simulink model "asm_blocks_lib"  (R2026b)
settings: Solver=VariableStepAuto
libraries: nesl_utility x45, asmlib_lib x25, fl_lib x3, ee_lib x3
(part 3 of 3)

== system asm_blocks_lib/Mechanik/Welle elastisch ==
  elastic_shaft : asmlib_lib/mechanics/Elastic shaft  c_W=c_W N*m/rad  d_W=d_W N*m*s/rad  t_specify=off  t_priority=None  t=0 N*m  t_nominal_specify=off  t_nominal_value=1  t_nominal_unit=N*m  w_specify=off  w_priority=None  w=0 rad/s  w_nominal_specify=off  w_nominal_value=1  w_nominal_unit=rad/s  phi_specify=off  phi_priority=High  phi=0 rad  phi_nominal_specify=off  phi_nominal_value=1  phi_nominal_unit=rad
  R : PMIOPort  Side=Left
  C : PMIOPort  Port=2  Side=Right
  connections:
  R/RConn1 -- elastic_shaft/LConn1
  C/RConn1 -- elastic_shaft/RConn1

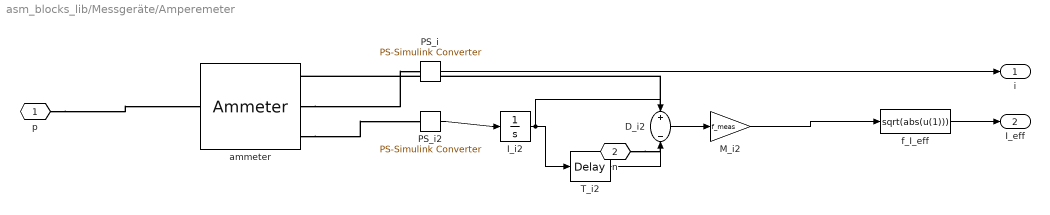
== system asm_blocks_lib/Messgeräte/Amperemeter ==
  D_i2 : Sum  Inputs=+-
  I_i2 : Integrator
  M_i2 : Gain  Gain=f_meas
  PS_i : nesl_utility/PS-Simulink Converter  PhysicalDomain=network_engine_domain  SubClassName=ps_output  LeftPortType=input  RightPortType=output  PseudoPeriodic=off  Frequencies=[]  VectorFormat=inherit  Unit=A  AffineConversion=off
  PS_i2 : nesl_utility/PS-Simulink Converter  PhysicalDomain=network_engine_domain  SubClassName=ps_output  LeftPortType=input  RightPortType=output  PseudoPeriodic=off  Frequencies=[]  VectorFormat=inherit  Unit=A^2  AffineConversion=off
  T_i2 : TransportDelay  DelayTime=1/f_meas  BufferSize=16384
  ammeter : asmlib_lib/sensors/Ammeter  ii_specify=off  ii_priority=None  ii=0 A  ii_nominal_specify=off  ii_nominal_value=1  ii_nominal_unit=A
  f_I_eff : Fcn  Expr=sqrt(abs(u(1)))
  p : PMIOPort  Side=Left
  n : PMIOPort  Port=2  Side=Right
  i : Outport
  I_eff : Outport  Port=2
  wires:
  PS_i/1 -> i/1
  PS_i2/1 -> I_i2/1
  I_i2/1 -> D_i2/1, T_i2/1
  T_i2/1 -> D_i2/2
  D_i2/1 -> M_i2/1
  M_i2/1 -> f_I_eff/1
  f_I_eff/1 -> I_eff/1
  connections:
  p/RConn1 -- ammeter/LConn1
  n/RConn1 -- ammeter/RConn1
  ammeter/RConn2 -- PS_i/LConn1
  ammeter/RConn3 -- PS_i2/LConn1

== system asm_blocks_lib/Messgeräte/Drehmomentmesswelle ==
  PS_M : nesl_utility/PS-Simulink Converter  PhysicalDomain=network_engine_domain  SubClassName=ps_output  LeftPortType=input  RightPortType=output  PseudoPeriodic=off  Frequencies=[]  VectorFormat=inherit  Unit=N*m  AffineConversion=off
  torque_sensor : asmlib_lib/sensors/Torque sensor  t_specify=off  t_priority=None  t=0 N*m  t_nominal_specify=off  t_nominal_value=1  t_nominal_unit=N*m
  R : PMIOPort  Side=Left
  C : PMIOPort  Port=2  Side=Right
  M : Outport
  wires:
  PS_M/1 -> M/1
  connections:
  R/RConn1 -- torque_sensor/LConn1
  C/RConn1 -- torque_sensor/RConn1
  torque_sensor/RConn2 -- PS_M/LConn1

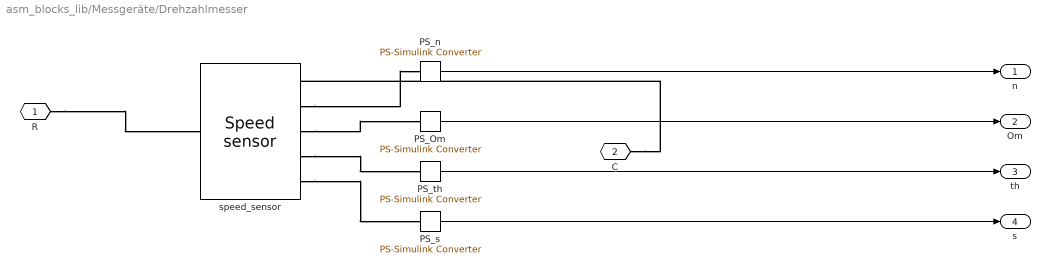
== system asm_blocks_lib/Messgeräte/Drehzahlmesser ==
  PS_Om : nesl_utility/PS-Simulink Converter  PhysicalDomain=network_engine_domain  SubClassName=ps_output  LeftPortType=input  RightPortType=output  PseudoPeriodic=off  Frequencies=[]  VectorFormat=inherit  Unit=rad/s  AffineConversion=off
  PS_n : nesl_utility/PS-Simulink Converter  PhysicalDomain=network_engine_domain  SubClassName=ps_output  LeftPortType=input  RightPortType=output  PseudoPeriodic=off  Frequencies=[]  VectorFormat=inherit  Unit=rpm  AffineConversion=off
  PS_s : nesl_utility/PS-Simulink Converter  PhysicalDomain=network_engine_domain  SubClassName=ps_output  LeftPortType=input  RightPortType=output  PseudoPeriodic=off  Frequencies=[]  VectorFormat=inherit  Unit=1  AffineConversion=off
  PS_th : nesl_utility/PS-Simulink Converter  PhysicalDomain=network_engine_domain  SubClassName=ps_output  LeftPortType=input  RightPortType=output  PseudoPeriodic=off  Frequencies=[]  VectorFormat=inherit  Unit=rad  AffineConversion=off
  speed_sensor : asmlib_lib/sensors/Speed sensor  ns=ns rpm  w_specify=off  w_priority=None  w=0 rad/s  w_nominal_specify=off  w_nominal_value=1  w_nominal_unit=rad/s  ph_specify=off  ph_priority=High  ph=0 rad  ph_nominal_specify=off  ph_nominal_value=1  ph_nominal_unit=rad
  R : PMIOPort  Side=Left
  C : PMIOPort  Port=2  Side=Right
  n : Outport
  Om : Outport  Port=2
  th : Outport  Port=3
  s : Outport  Port=4
  wires:
  PS_n/1 -> n/1
  PS_Om/1 -> Om/1
  PS_th/1 -> th/1
  PS_s/1 -> s/1
  connections:
  R/RConn1 -- speed_sensor/LConn1
  C/RConn1 -- speed_sensor/RConn1
  speed_sensor/RConn2 -- PS_n/LConn1
  speed_sensor/RConn3 -- PS_Om/LConn1
  speed_sensor/RConn4 -- PS_th/LConn1
  speed_sensor/RConn5 -- PS_s/LConn1

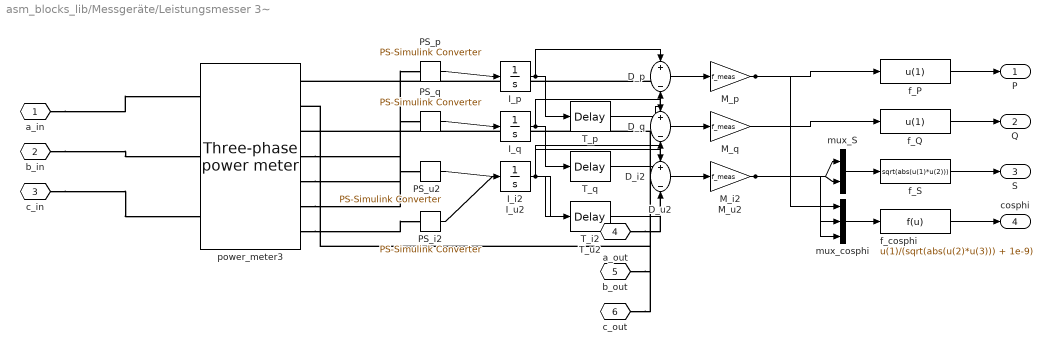
== system asm_blocks_lib/Messgeräte/Leistungsmesser 3~ ==
  D_i2 : Sum  Inputs=+-
  D_p : Sum  Inputs=+-
  D_q : Sum  Inputs=+-
  D_u2 : Sum  Inputs=+-
  I_i2 : Integrator
  I_p : Integrator
  I_q : Integrator
  I_u2 : Integrator
  M_i2 : Gain  Gain=f_meas
  M_p : Gain  Gain=f_meas
  M_q : Gain  Gain=f_meas
  M_u2 : Gain  Gain=f_meas
  PS_i2 : nesl_utility/PS-Simulink Converter  PhysicalDomain=network_engine_domain  SubClassName=ps_output  LeftPortType=input  RightPortType=output  PseudoPeriodic=off  Frequencies=[]  VectorFormat=inherit  Unit=A^2  AffineConversion=off
  PS_p : nesl_utility/PS-Simulink Converter  PhysicalDomain=network_engine_domain  SubClassName=ps_output  LeftPortType=input  RightPortType=output  PseudoPeriodic=off  Frequencies=[]  VectorFormat=inherit  Unit=W  AffineConversion=off
  PS_q : nesl_utility/PS-Simulink Converter  PhysicalDomain=network_engine_domain  SubClassName=ps_output  LeftPortType=input  RightPortType=output  PseudoPeriodic=off  Frequencies=[]  VectorFormat=inherit  Unit=V*A  AffineConversion=off
  PS_u2 : nesl_utility/PS-Simulink Converter  PhysicalDomain=network_engine_domain  SubClassName=ps_output  LeftPortType=input  RightPortType=output  PseudoPeriodic=off  Frequencies=[]  VectorFormat=inherit  Unit=V^2  AffineConversion=off
  T_i2 : TransportDelay  DelayTime=1/f_meas  BufferSize=16384
  T_p : TransportDelay  DelayTime=1/f_meas  BufferSize=16384
  T_q : TransportDelay  DelayTime=1/f_meas  BufferSize=16384
  T_u2 : TransportDelay  DelayTime=1/f_meas  BufferSize=16384
  f_P : Fcn  Expr=u(1)
  f_Q : Fcn  Expr=u(1)
  f_S : Fcn  Expr=sqrt(abs(u(1)*u(2)))
  f_cosphi : Fcn  Expr=u(1)/(sqrt(abs(u(2)*u(3))) + 1e-9)
  mux_S : Mux  Inputs=2
  mux_cosphi : Mux  Inputs=3
  power_meter3 : asmlib_lib/sensors/Three-phase power meter  ia_specify=off  ia_priority=None  ia=0 A  ia_nominal_specify=off  ia_nominal_value=1  ia_nominal_unit=A  ib_specify=off  ib_priority=None  ib=0 A  ib_nominal_specify=off  ib_nominal_value=1  ib_nominal_unit=A  ic_specify=off  ic_priority=None  ic=0 A  ic_nominal_specify=off  ic_nominal_value=1  ic_nominal_unit=A
  a_in : PMIOPort  Side=Left
  b_in : PMIOPort  Port=2  Side=Left
  c_in : PMIOPort  Port=3  Side=Left
  a_out : PMIOPort  Port=4  Side=Right
  b_out : PMIOPort  Port=5  Side=Right
  c_out : PMIOPort  Port=6  Side=Right
  P : Outport
  Q : Outport  Port=2
  S : Outport  Port=3
  cosphi : Outport  Port=4
  wires:
  PS_p/1 -> I_p/1
  I_p/1 -> D_p/1, T_p/1
  T_p/1 -> D_p/2
  D_p/1 -> M_p/1
  M_p/1 -> f_P/1, mux_cosphi/1
  f_P/1 -> P/1
  PS_q/1 -> I_q/1
  I_q/1 -> D_q/1, T_q/1
  T_q/1 -> D_q/2
  D_q/1 -> M_q/1
  M_q/1 -> f_Q/1
  f_Q/1 -> Q/1
  PS_u2/1 -> I_u2/1
  I_u2/1 -> D_u2/1, T_u2/1
  T_u2/1 -> D_u2/2
  D_u2/1 -> M_u2/1
  PS_i2/1 -> I_i2/1
  I_i2/1 -> D_i2/1, T_i2/1
  T_i2/1 -> D_i2/2
  D_i2/1 -> M_i2/1
  M_u2/1 -> mux_S/1, mux_cosphi/2
  M_i2/1 -> mux_S/2, mux_cosphi/3
  mux_S/1 -> f_S/1
  f_S/1 -> S/1
  mux_cosphi/1 -> f_cosphi/1
  f_cosphi/1 -> cosphi/1
  connections:
  a_in/RConn1 -- power_meter3/LConn1
  b_in/RConn1 -- power_meter3/LConn2
  c_in/RConn1 -- power_meter3/LConn3
  a_out/RConn1 -- power_meter3/RConn1
  b_out/RConn1 -- power_meter3/RConn2
  c_out/RConn1 -- power_meter3/RConn3
  power_meter3/RConn4 -- PS_p/LConn1
  power_meter3/RConn5 -- PS_q/LConn1
  power_meter3/RConn6 -- PS_u2/LConn1
  power_meter3/RConn7 -- PS_i2/LConn1

== system asm_blocks_lib/Messgeräte/Luftspalt-Sonde ==
  PS_Bhat : nesl_utility/PS-Simulink Converter  PhysicalDomain=network_engine_domain  SubClassName=ps_output  LeftPortType=input  RightPortType=output  PseudoPeriodic=off  Frequencies=[]  VectorFormat=inherit  Unit=T  AffineConversion=off
  PS_psi_h : nesl_utility/PS-Simulink Converter  PhysicalDomain=network_engine_domain  SubClassName=ps_output  LeftPortType=input  RightPortType=output  PseudoPeriodic=off  Frequencies=[]  VectorFormat=inherit  Unit=Wb  AffineConversion=off
  airgap_probe : asmlib_lib/sensors/Air-gap probe  p=p  N1xi1=N1xi1  l=l m  r=r m  psih_specify=off  psih_priority=None  psih=zeros(2, 1) Wb  psih_nominal_specify=off  psih_nominal_value=1  psih_nominal_unit=Wb
  f_phi_el : Fcn  Expr=atan2(u(2),u(1))
  LS : PMIOPort  Side=Left
  psi_h : Outport
  phi_el : Outport  Port=2
  Bhat : Outport  Port=3
  wires:
  PS_psi_h/1 -> psi_h/1, f_phi_el/1
  f_phi_el/1 -> phi_el/1
  PS_Bhat/1 -> Bhat/1
  connections:
  LS/RConn1 -- airgap_probe/LConn1
  airgap_probe/RConn1 -- PS_psi_h/LConn1
  airgap_probe/RConn2 -- PS_Bhat/LConn1

== system asm_blocks_lib/Messgeräte/Schreiber ==
  u : Inport
  Scope : Scope
  wires:
  u/1 -> Scope/1

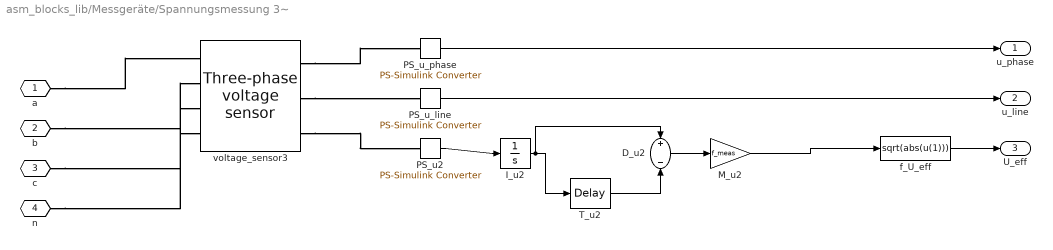
== system asm_blocks_lib/Messgeräte/Spannungsmessung 3~ ==
  D_u2 : Sum  Inputs=+-
  I_u2 : Integrator
  M_u2 : Gain  Gain=f_meas
  PS_u2 : nesl_utility/PS-Simulink Converter  PhysicalDomain=network_engine_domain  SubClassName=ps_output  LeftPortType=input  RightPortType=output  PseudoPeriodic=off  Frequencies=[]  VectorFormat=inherit  Unit=V^2  AffineConversion=off
  PS_u_line : nesl_utility/PS-Simulink Converter  PhysicalDomain=network_engine_domain  SubClassName=ps_output  LeftPortType=input  RightPortType=output  PseudoPeriodic=off  Frequencies=[]  VectorFormat=inherit  Unit=V  AffineConversion=off
  PS_u_phase : nesl_utility/PS-Simulink Converter  PhysicalDomain=network_engine_domain  SubClassName=ps_output  LeftPortType=input  RightPortType=output  PseudoPeriodic=off  Frequencies=[]  VectorFormat=inherit  Unit=V  AffineConversion=off
  T_u2 : TransportDelay  DelayTime=1/f_meas  BufferSize=16384
  f_U_eff : Fcn  Expr=sqrt(abs(u(1)))
  voltage_sensor3 : asmlib_lib/sensors/Three-phase voltage sensor  reference=reference
  a : PMIOPort  Side=Left
  b : PMIOPort  Port=2  Side=Left
  c : PMIOPort  Port=3  Side=Left
  n : PMIOPort  Port=4  Side=Left
  u_phase : Outport
  u_line : Outport  Port=2
  U_eff : Outport  Port=3
  wires:
  PS_u_phase/1 -> u_phase/1
  PS_u_line/1 -> u_line/1
  PS_u2/1 -> I_u2/1
  I_u2/1 -> D_u2/1, T_u2/1
  T_u2/1 -> D_u2/2
  D_u2/1 -> M_u2/1
  M_u2/1 -> f_U_eff/1
  f_U_eff/1 -> U_eff/1
  connections:
  a/RConn1 -- voltage_sensor3/LConn1
  b/RConn1 -- voltage_sensor3/LConn2
  c/RConn1 -- voltage_sensor3/LConn3
  n/RConn1 -- voltage_sensor3/LConn4
  voltage_sensor3/RConn1 -- PS_u_phase/LConn1
  voltage_sensor3/RConn2 -- PS_u_line/LConn1
  voltage_sensor3/RConn3 -- PS_u2/LConn1

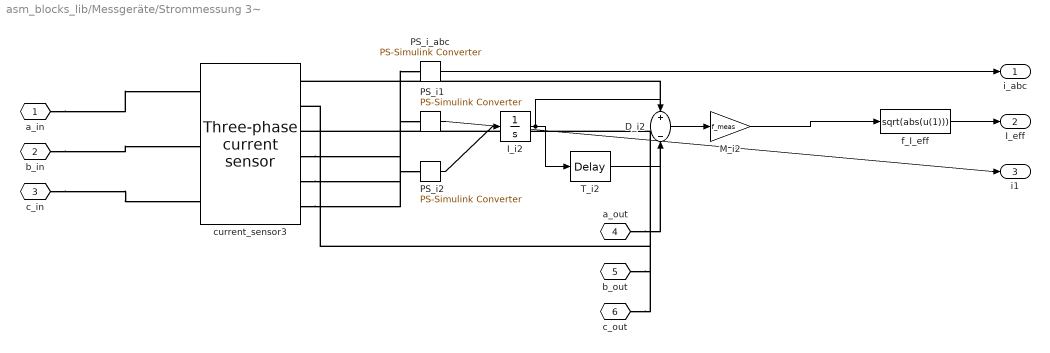
== system asm_blocks_lib/Messgeräte/Strommessung 3~ ==
  D_i2 : Sum  Inputs=+-
  I_i2 : Integrator
  M_i2 : Gain  Gain=f_meas
  PS_i1 : nesl_utility/PS-Simulink Converter  PhysicalDomain=network_engine_domain  SubClassName=ps_output  LeftPortType=input  RightPortType=output  PseudoPeriodic=off  Frequencies=[]  VectorFormat=inherit  Unit=A  AffineConversion=off
  PS_i2 : nesl_utility/PS-Simulink Converter  PhysicalDomain=network_engine_domain  SubClassName=ps_output  LeftPortType=input  RightPortType=output  PseudoPeriodic=off  Frequencies=[]  VectorFormat=inherit  Unit=A^2  AffineConversion=off
  PS_i_abc : nesl_utility/PS-Simulink Converter  PhysicalDomain=network_engine_domain  SubClassName=ps_output  LeftPortType=input  RightPortType=output  PseudoPeriodic=off  Frequencies=[]  VectorFormat=inherit  Unit=A  AffineConversion=off
  T_i2 : TransportDelay  DelayTime=1/f_meas  BufferSize=16384
  current_sensor3 : asmlib_lib/sensors/Three-phase current sensor  ia_specify=off  ia_priority=None  ia=0 A  ia_nominal_specify=off  ia_nominal_value=1  ia_nominal_unit=A  ib_specify=off  ib_priority=None  ib=0 A  ib_nominal_specify=off  ib_nominal_value=1  ib_nominal_unit=A  ic_specify=off  ic_priority=None  ic=0 A  ic_nominal_specify=off  ic_nominal_value=1  ic_nominal_unit=A
  f_I_eff : Fcn  Expr=sqrt(abs(u(1)))
  a_in : PMIOPort  Side=Left
  b_in : PMIOPort  Port=2  Side=Left
  c_in : PMIOPort  Port=3  Side=Left
  a_out : PMIOPort  Port=4  Side=Right
  b_out : PMIOPort  Port=5  Side=Right
  c_out : PMIOPort  Port=6  Side=Right
  i_abc : Outport
  I_eff : Outport  Port=2
  i1 : Outport  Port=3
  wires:
  PS_i_abc/1 -> i_abc/1
  PS_i2/1 -> I_i2/1
  I_i2/1 -> D_i2/1, T_i2/1
  T_i2/1 -> D_i2/2
  D_i2/1 -> M_i2/1
  M_i2/1 -> f_I_eff/1
  f_I_eff/1 -> I_eff/1
  PS_i1/1 -> i1/1
  connections:
  a_in/RConn1 -- current_sensor3/LConn1
  b_in/RConn1 -- current_sensor3/LConn2
  c_in/RConn1 -- current_sensor3/LConn3
  a_out/RConn1 -- current_sensor3/RConn1
  b_out/RConn1 -- current_sensor3/RConn2
  c_out/RConn1 -- current_sensor3/RConn3
  current_sensor3/RConn4 -- PS_i_abc/LConn1
  current_sensor3/RConn5 -- PS_i1/LConn1
  current_sensor3/RConn6 -- PS_i2/LConn1

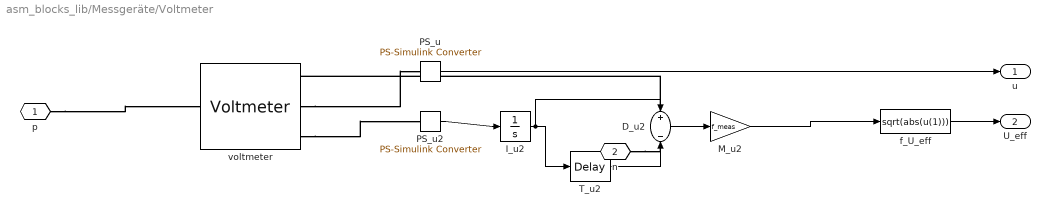
== system asm_blocks_lib/Messgeräte/Voltmeter ==
  D_u2 : Sum  Inputs=+-
  I_u2 : Integrator
  M_u2 : Gain  Gain=f_meas
  PS_u : nesl_utility/PS-Simulink Converter  PhysicalDomain=network_engine_domain  SubClassName=ps_output  LeftPortType=input  RightPortType=output  PseudoPeriodic=off  Frequencies=[]  VectorFormat=inherit  Unit=V  AffineConversion=off
  PS_u2 : nesl_utility/PS-Simulink Converter  PhysicalDomain=network_engine_domain  SubClassName=ps_output  LeftPortType=input  RightPortType=output  PseudoPeriodic=off  Frequencies=[]  VectorFormat=inherit  Unit=V^2  AffineConversion=off
  T_u2 : TransportDelay  DelayTime=1/f_meas  BufferSize=16384
  f_U_eff : Fcn  Expr=sqrt(abs(u(1)))
  voltmeter : asmlib_lib/sensors/Voltmeter
  p : PMIOPort  Side=Left
  n : PMIOPort  Port=2  Side=Right
  u : Outport
  U_eff : Outport  Port=2
  wires:
  PS_u/1 -> u/1
  PS_u2/1 -> I_u2/1
  I_u2/1 -> D_u2/1, T_u2/1
  T_u2/1 -> D_u2/2
  D_u2/1 -> M_u2/1
  M_u2/1 -> f_U_eff/1
  f_U_eff/1 -> U_eff/1
  connections:
  p/RConn1 -- voltmeter/LConn1
  n/RConn1 -- voltmeter/RConn1
  voltmeter/RConn2 -- PS_u/LConn1
  voltmeter/RConn3 -- PS_u2/LConn1

== system asm_blocks_lib/Quellen/Netz 3~ ==
  grid3 : asmlib_lib/sources/Three-phase grid  U_L=U_L V  f1=f1 Hz  phase_seq=phase_seq  phi0=phi0 deg  t_on=t_on s  R_N=R_N Ohm  L_N=L_N H  ia_specify=off  ia_priority=None  ia=0 A  ia_nominal_specify=off  ia_nominal_value=1  ia_nominal_unit=A  ib_specify=off  ib_priority=None  ib=0 A  ib_nominal_specify=off  ib_nominal_value=1  ib_nominal_unit=A  ic_specify=off  ic_priority=None  ic=0 A  ic_nominal_specify=off  ic_nominal_value=1  ic_nominal_unit=A
  a : PMIOPort  Side=Right
  b : PMIOPort  Port=2  Side=Right
  c : PMIOPort  Port=3  Side=Right
  n : PMIOPort  Port=4  Side=Right
  connections:
  a/RConn1 -- grid3/RConn1
  b/RConn1 -- grid3/RConn2
  c/RConn1 -- grid3/RConn3
  n/RConn1 -- grid3/RConn4

== system asm_blocks_lib/Quellen/Sternpunkt (Erde) ==
  neutral_ground : fl_lib/Electrical/Electrical Elements/Electrical Reference
  N : PMIOPort  Side=Left
  connections:
  N/RConn1 -- neutral_ground/LConn1

== system asm_blocks_lib/Referenz/ASM Kloss (quasistationär) ==
  PS_M : nesl_utility/PS-Simulink Converter  PhysicalDomain=network_engine_domain  SubClassName=ps_output  LeftPortType=input  RightPortType=output  PseudoPeriodic=off  Frequencies=[]  VectorFormat=inherit  Unit=N*m  AffineConversion=off
  PS_s : nesl_utility/PS-Simulink Converter  PhysicalDomain=network_engine_domain  SubClassName=ps_output  LeftPortType=input  RightPortType=output  PseudoPeriodic=off  Frequencies=[]  VectorFormat=inherit  Unit=1  AffineConversion=off
  asm_kloss : asmlib_lib/reference/ASM Kloss (quasi-static)  MK=MK N*m  sK=sK  ns=ns rpm  t_specify=off  t_priority=None  t=0 N*m  t_nominal_specify=off  t_nominal_value=1  t_nominal_unit=N*m  w_specify=off  w_priority=None  w=0 rad/s  w_nominal_specify=off  w_nominal_value=1  w_nominal_unit=rad/s  sl_specify=off  sl_priority=None  sl=0  sl_nominal_specify=off  sl_nominal_value=1  sl_nominal_unit=1
  R : PMIOPort  Side=Right
  C : PMIOPort  Port=2  Side=Right
  M : Outport
  s : Outport  Port=2
  wires:
  PS_M/1 -> M/1
  PS_s/1 -> s/1
  connections:
  R/RConn1 -- asm_kloss/RConn1
  C/RConn1 -- asm_kloss/RConn2
  asm_kloss/RConn3 -- PS_M/LConn1
  asm_kloss/RConn4 -- PS_s/LConn1

== system asm_blocks_lib/Referenz/ASM Referenz (Simscape Electrical) ==
  J_M : fl_lib/Mechanical/Rotational Elements/Inertia  inertia=J_M kg*m^2  num_ports=foundation.enum.numPorts2.one  w_specify=off  w_priority=High  w=0 rad/s  w_nominal_specify=off  w_nominal_value=1  w_nominal_unit=rad/s  t_specify=off  t_priority=None  t=0 N*m  t_nominal_specify=off  t_nominal_value=1  t_nominal_unit=N*m
  Leiter : ee_lib/Connectors & References/Phase Splitter
  Maschine : ee_lib/Electromechanical/Asynchronous/Induction Machine Squirrel Cage  port_option=ee.enum.threePhasePort.composite  SRated=sqrt(3)*U_N*10 A*V  VRated=U_N V  FRated=f_N Hz  nPolePairs=p  param_unit=ee.enum.unit.si  squirrel_cage=ee.enum.squirrelcage.Single  zero_sequence=ee.enum.park.zerosequence.include  initialization_option=ee.enum.asm.initialization.fluxvariables  Rs=R1 Ohm  Xls=2*pi*f_N*L1s Ohm  pu_Rs=0.0258  pu_Lls=0.0413  Rrd=R2b Ohm  Xlrd=2*pi*f_N*L2sb Ohm  pu_Rrd=0.0145  pu_Llrd=0.0424  Rrd1=0.28 Ohm  Xlrd1=0.82 Ohm  Rrd2=0.28 Ohm  Xlrd2=0.82 Ohm  pu_Rrd1=0.0290  pu_Llrd1=0.0848  pu_Rrd2=0.0290  pu_Llrd2=0.0848  Xm=2*pi*f_N*Lh Ohm  pu_Lm=1.7562  X0=2*pi*f_N*L1s Ohm  pu_L0=0.0413  saturation_option=ee.enum.saturation.exclude  saturation_i=[0, 4, 9, 18, 25, 34, 50, 68, 95, 120] A  saturation_v=[0, 88, 154, 198, 220, 242, 264, 286, 308, 327] V  pu_saturation_i=[0, .176, .396, .792, 1.1, 1.496, 2.2, 2.992, 4.18, 5.28]  pu_saturation_v=[0, .4, .7, .9, 1, 1.1, 1.2, 1.3, 1.4, 1.4864]  connection_option=ee.enum.Connection.delta  angular_position_specify=off  angular_position_priority=None  angular_position=0 deg  angular_position_nominal_specify=off  angular_position_nominal_value=1  angular_position_nominal_unit=deg  pu_psids_specify=off  pu_psids_priority=None  pu_psids=0  pu_psids_nominal_specify=off  pu_psids_nominal_value=1  pu_psids_nominal_unit=1  pu_psiqs_specify=off  pu_psiqs_priority=None  pu_psiqs=0  pu_psiqs_nominal_specify=off  pu_psiqs_nominal_value=1  pu_psiqs_nominal_unit=1  pu_psi0s_specify=off  pu_psi0s_priority=None  pu_psi0s=0  pu_psi0s_nominal_specify=off  pu_psi0s_nominal_value=1  pu_psi0s_nominal_unit=1  pu_psidr_specify=off  pu_psidr_priority=None  pu_psidr=0  pu_psidr_nominal_specify=off  pu_psidr_nominal_value=1  pu_psidr_nominal_unit=1  pu_psiqr_specify=off  pu_psiqr_priority=None  pu_psiqr=0  pu_psiqr_nominal_specify=off  pu_psiqr_nominal_value=1  pu_psiqr_nominal_unit=1  pu_psidr1_specify=off  pu_psidr1_priority=None  pu_psidr1=0  pu_psidr1_nominal_specify=off  pu_psidr1_nominal_value=1  pu_psidr1_nominal_unit=1  pu_psiqr1_specify=off  pu_psiqr1_priority=None  pu_psiqr1=0  pu_psiqr1_nominal_specify=off  pu_psiqr1_nominal_value=1  pu_psiqr1_nominal_unit=1  pu_psidr2_specify=off  pu_psidr2_priority=None  pu_psidr2=0  pu_psidr2_nominal_specify=off  pu_psidr2_nominal_value=1  pu_psidr2_nominal_unit=1  pu_psiqr2_specify=off  pu_psiqr2_priority=None  pu_psiqr2=0  pu_psiqr2_nominal_specify=off  pu_psiqr2_nominal_value=1  pu_psiqr2_nominal_unit=1  psids_specify=on  psids_priority=High  psids=0 Wb  psids_nominal_specify=off  psids_nominal_value=1  psids_nominal_unit=Wb  psiqs_specify=on  psiqs_priority=High  psiqs=0 Wb  psiqs_nominal_specify=off  psiqs_nominal_value=1  psiqs_nominal_unit=Wb  psi0s_specify=off  psi0s_priority=None  psi0s=0 Wb  psi0s_nominal_specify=off  psi0s_nominal_value=1  psi0s_nominal_unit=Wb  psidr_specify=on  psidr_priority=High  psidr=0 Wb  psidr_nominal_specify=off  psidr_nominal_value=1  psidr_nominal_unit=Wb  psiqr_specify=on  psiqr_priority=High  psiqr=0 Wb  psiqr_nominal_specify=off  psiqr_nominal_value=1  psiqr_nominal_unit=Wb  psidr1_specify=off  psidr1_priority=None  psidr1=0 Wb  psidr1_nominal_specify=off  psidr1_nominal_value=1  psidr1_nominal_unit=Wb  psiqr1_specify=off  psiqr1_priority=None  psiqr1=0 Wb  psiqr1_nominal_specify=off  psiqr1_nominal_value=1  psiqr1_nominal_unit=Wb  psidr2_specify=off  psidr2_priority=None  psidr2=0 Wb  psidr2_nominal_specify=off  psidr2_nominal_value=1  psidr2_nominal_unit=Wb  psiqr2_specify=off  psiqr2_priority=None  psiqr2=0 Wb  psiqr2_nominal_specify=off  psiqr2_nominal_value=1  psiqr2_nominal_unit=Wb  slip_specify=off  slip_priority=None  slip=0  slip_nominal_specify=off  slip_nominal_value=1  slip_nominal_unit=1  real_power_generated_specify=off  real_power_generated_priority=None  real_power_generated=0 W  real_power_generated_nominal_specify=off  real_power_generated_nominal_value=1  real_power_generated_nominal_unit=W  mechanical_power_consumed_specify=off  mechanical_power_consumed_priority=None  mechanical_power_consumed=0 W  mechanical_power_consumed_nominal_specify=off  mechanical_power_consumed_nominal_value=1  mechanical_power_consumed_nominal_unit=W  Tmeas=298.15 K  alpha=3.93e-3 1/K  alpha_cage=4.4e-3 1/K  stator_thermal_mass=100 J/K  rotor_thermal_mass=200 J/K  temperatureA_specify=off  temperatureA_priority=High  temperatureA=25 degC  temperatureA_nominal_specify=off  temperatureA_nominal_value=1  temperatureA_nominal_unit=degC  temperatureB_specify=off  temperatureB_priority=High  temperatureB=25 degC  temperatureB_nominal_specify=off  temperatureB_nominal_value=1  temperatureB_nominal_unit=degC  temperatureC_specify=off  temperatureC_priority=High  temperatureC=25 degC  temperatureC_nominal_specify=off  temperatureC_nominal_value=1  temperatureC_nominal_unit=degC  temperatureR_specify=off  temperatureR_priority=High  temperatureR=25 degC  temperatureR_nominal_specify=off  temperatureR_nominal_value=1  temperatureR_nominal_unit=degC
  Sternpunkt : ee_lib/Connectors & References/Floating Neutral (Three-Phase)  port_option=ee.enum.threePhasePort.composite  G_parasitic=1e-12 1/Ohm
  a : PMIOPort  Side=Left
  b : PMIOPort  Port=2  Side=Left
  c : PMIOPort  Port=3  Side=Left
  R : PMIOPort  Port=4  Side=Right
  C : PMIOPort  Port=5  Side=Right
  connections:
  a/RConn1 -- Leiter/RConn1
  b/RConn1 -- Leiter/RConn2
  c/RConn1 -- Leiter/RConn3
  Leiter/LConn1 -- Maschine/RConn2
  Maschine/RConn3 -- Sternpunkt/LConn1
  Maschine/LConn1 -- R/RConn1 -- J_M/LConn1
  C/RConn1 -- Maschine/LConn2

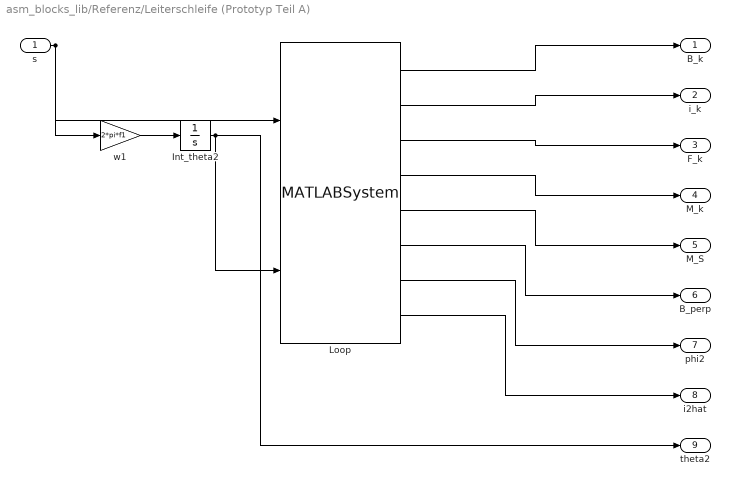
== system asm_blocks_lib/Referenz/Leiterschleife (Prototyp Teil A) ==
  s : Inport
  Int_theta2 : Integrator
  Loop : MATLABSystem  System=asmtools.ConductorLoop  Bhat=Bhat  l=l  r=r  f1=f1  p=p  R2_S=R2_S  L2s_S=L2s_S  conv=3 - 2*conv_phi2  mode=phi2_mode  phi2_fix=phi2_fix  SimulateUsing=Interpreted execution
      mask Type: asmtools.ConductorLoop
  w1 : Gain  Gain=2*pi*f1
  B_k : Outport
  i_k : Outport  Port=2
  F_k : Outport  Port=3
  M_k : Outport  Port=4
  M_S : Outport  Port=5
  B_perp : Outport  Port=6
  phi2 : Outport  Port=7
  i2hat : Outport  Port=8
  theta2 : Outport  Port=9
  wires:
  s/1 -> w1/1, Loop/1
  w1/1 -> Int_theta2/1
  Int_theta2/1 -> Loop/2, theta2/1
  Loop/1 -> B_k/1
  Loop/2 -> i_k/1
  Loop/3 -> F_k/1
  Loop/4 -> M_k/1
  Loop/5 -> M_S/1
  Loop/6 -> B_perp/1
  Loop/7 -> phi2/1
  Loop/8 -> i2hat/1
